simulink model "Cascaded_Rectifier_Isolated_Output"  (R2021b)
settings: Solver=VariableStepAuto  StartTime=0.0  StopTime=0.5  RelTol=1e-3
libraries: spsSeriesRLCBranchLib x41, spsUniversalBridgeLib x28, spsVoltageMeasurementLib x18, spsLinearTransformerLib x8, simulink x8, spsThreeLevelBridgeLib x7, spsACVoltageSourceLib x1, spsCurrentMeasurementLib x1, spsMeanLib x1, slpidlib x1, powerlib_extras x1, spsTHDLib x1
(part 1 of 2)
settings Model: SimulationMode=accelerator  Creator=abc6820292  LastModifiedBy=abc68
settings SolverCC: ZeroCrossAlgorithm=Adaptive
settings DataIOCC: ReturnWorkspaceOutputs=off  Refine=10
settings DebuggingCC: MaskedZcDiagnostic=none  IgnoredZcDiagnostic=none

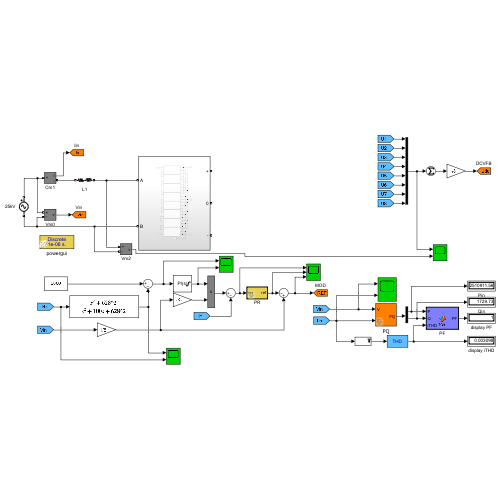
[thumbnail: Simulink's stored preview of the top-level diagram]
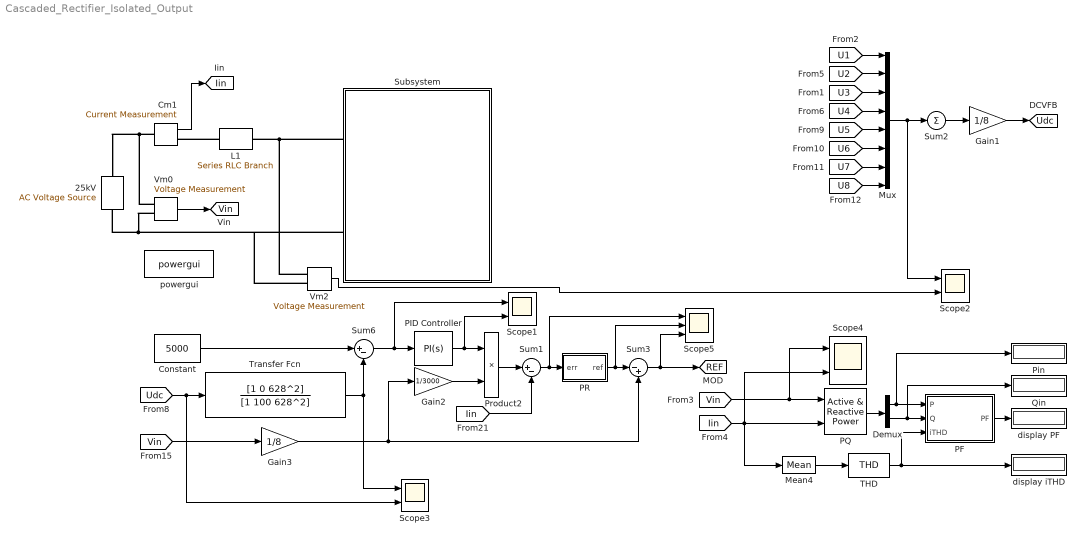
== system Cascaded_Rectifier_Isolated_Output ==
  25kV : spsACVoltageSourceLib/AC Voltage Source  Amplitude=37000  Phase=0  Frequency=50  SampleTime=0  Measurements=None  BusType=swing  Pref=10e3  Qref=0  Qmin=-inf  Qmax=+inf
  Cm1 : spsCurrentMeasurementLib/Current Measurement  PhasorSimulation=off  OutputType=Complex  PSBequivalent=0
  Constant : Constant  Value=5000
  Demux : Demux  Outputs=2
  Gain1 : Gain  Gain=1/8
  Gain2 : Gain  Gain=1/3000
  Gain3 : Gain  Gain=1/8
  L1 : spsSeriesRLCBranchLib/Series RLC Branch  LConnTagsString=__new0  RConnTagsString=__new0  BranchType=RL  Resistance=0.01  Inductance=0.01  SetiL0=off  InitialCurrent=0  Capacitance=inf  Setx0=off  InitialVoltage=0  Measurements=None
  Mean4 : spsMeanLib/Mean  Freq=5000  Vinit=0  Ts=0
  Mux : Mux  Inputs=8
  PF : MATLAB Function  TreatAsAtomicUnit=on
  PID Controller : slpidlib/PID Controller  Controller=PI  Form=Parallel  TimeDomain=Continuous-time  UseExternalTs=off  SampleTime=-1  IntegratorMethod=Forward Euler  FilterMethod=Forward Euler  ControllerParametersSource=internal  P=0.08  I=8  D=0.005  UseFilter=on  N=100  TunerSelectOption=Transfer Function Based (PID Tuner App)  InitialConditionSource=internal  InitialConditionForIntegrator=0  InitialConditionForFilter=0  DifferentiatorICPrevScaledInput=0  ExternalReset=none  TrackingMode=off  Kt=1  LimitOutput=on  SatLimitsSource=internal  UpperSaturationLimit=400  LowerSaturationLimit=-400  LinearizeAsGain=on  AntiWindupMode=clamping  Kb=1  POutMin=[]  POutMax=[]  IOutMin=[]  IOutMax=[]  DOutMin=[]  DOutMax=[]  NOutMin=[]  NOutMax=[]  SumOutMin=[]  SumOutMax=[]  SaturationOutMin=[]  SaturationOutMax=[]  PParamMin=[]  PParamMax=[]  IParamMin=[]  IParamMax=[]  DParamMin=[]  DParamMax=[]  NParamMin=[]  NParamMax=[]  KbParamMin=[]  KbParamMax=[]  KtParamMin=[]  KtParamMax=[]  KbOutMin=[]  KbOutMax=[]  KtOutMin=[]  KtOutMax=[]  IntegratorOutMin=[]  IntegratorOutMax=[]  FilterOutMin=[]  FilterOutMax=[]  SumI1OutMin=[]  SumI1OutMax=[]  SumI2OutMin=[]  SumI2OutMax=[]  SumI3OutMin=[]  SumI3OutMax=[]  SumI4OutMin=[]  SumI4OutMax=[]  SumDOutMin=[]  SumDOutMax=[]  DifferentiatorOutMin=[]  DifferentiatorOutMax=[]  FilterDiffOutCoefMin=[]  FilterDiffOutCoefMax=[]  ReciprocalOutMin=[]  ReciprocalOutMax=[]  SumDenOutMin=[]  SumDenOutMax=[]  SumNumOutMin=[]  SumNumOutMax=[]  DivideOutMin=[]  DivideOutMax=[]  UdiffTsProdOutMin=[]  UdiffTsProdOutMax=[]  NTsProdOutMin=[]  NTsProdOutMax=[]  UintegralTsProdOutMin=[]  UintegralTsProdOutMax=[]  UngainTsProdOutMin=[]  UngainTsProdOutMax=[]  FilterDenConstantOutDataTypeStr=Inherit: Inherit via back propagation  FilterDenConstantOutMin=[]  FilterDenConstantOutMax=[]  PCopyOutDataTypeStr=Inherit: Inherit via back propagation  PCopyOutMin=[]  PCopyOutMax=[]  NCopyOutDataTypeStr=Inherit: Inherit via back propagation  NCopyOutMin=[]  NCopyOutMax=[]  IntegratorContinuousStateAttributes=''  IntegratorStateMustResolveToSignalObject=off  IntegratorRTWStateStorageClass=Auto  FilterContinuousStateAttributes=''  FilterStateMustResolveToSignalObject=off  FilterRTWStateStorageClass=Auto  ParallelPVariant=InternalParameters  IdealPVariant=Disabled  IVariant=InternalParameters  DVariant=Disabled  IntegratorVariant=Continuous  SatVariant=Enabled  AWVariant=ContClampingParallel  PCopyVariant=Disabled  TRVariant=Disabled  FdbkBlocksVariant=Forward  IdealPFdbkVariant=Disabled  SatFdbkVariant=Disabled  DerivativeFilterVariant=Disabled  NVariant=Disabled  NCopyVariant=Disabled_SignalSpec  FilterICVariant=Disabled  IntegratorICVariant=InternalICs  ExternalResetVariant=Disabled  TRSumVariant=Passthrough  SumFdbkVariant=Disabled  SumVariant=Sum_PI  TsampFilterVariant=InternalTs  TsampNgainVariant=Passthrough  TsampIntegralVariant=Passthrough  ExternalSaturationOutDataTypeStr=Inherit: Same as second input
  PQ : powerlib_extras/Measurements/Active & Reactive Power  f1=50
      settings: SourceProductBaseCode=PS
  PR : Subsystem  TreatAsAtomicUnit=on  mask{Kp=12, Kr=1000, Wc=5, Upper=5000, Lower=-5000}
  Pin : Display
      settings: Format=bank
  Product2 : Product  RndMeth=Zero
  Qin : Display
      settings: Format=bank
  Scope{1..4} (4 alike) : Scope  NumInputPorts=2
  Scope5 : Scope  NumInputPorts=3
  Subsystem : Subsystem
  Sum1 : Sum  Inputs=|+-
  Sum2 : Sum  Inputs=+
  Sum3 : Sum  Inputs=|-+
  Sum6 : Sum  Inputs=|+-
  THD : spsTHDLib/THD  Freq=50  Ts=0
      settings: SourceProductBaseCode=PS
  Transfer Fcn : TransferFcn  Numerator=[1 0 628^2]  Denominator=[1 100 628^2]
  Vm0 : spsVoltageMeasurementLib/Voltage Measurement  PhasorSimulation=off  OutputType=Complex  PSBequivalent=0
  Vm2 : spsVoltageMeasurementLib/Voltage Measurement  PhasorSimulation=off  OutputType=Complex  PSBequivalent=0
  display PF : Display
  display iTHD : Display
  powergui : spspowerguiLib/powergui  SimulationMode=Discrete  SampleTime=1e-6  frequency=60  Iterations=50  frequencyindice=0  Pbase=100e6  ErrMax=1e-4  UnitsV=kV  UnitsW=MW  buscounter=0  FunctionMessages=off  echomessages=off  EnableUseOfTLC=off  CurrentSourceSwitches=off  DisableSnubberDevices=off  DisableRonSwitches=off  DisableVfSwitches=off  DisplayEquations=off  AutomaticDiscreteSolvers=off  SolverType=Tustin/Backward Euler (TBE)  Interpol=off  ExternalGateDelay=off  methode=off  Ts=0  x0status=blocks  SPID=off  SwTol=0  HookPort=off  NonlinearTolerance=1e-4  nMaxIteration=100  ContinueOnMaxIteration=off  RestoreLinks=warning  ResistiveCurrentMeasurement=off  Frange=[0:2:500]  Ylog=off  Xlog=on  ShowGrid=off  save=off  variable=ZData  structure=QQQQQ  ZoomFFT=off  StartTime=0.5  cycles=15  DisplayStyle=1  fundamental=50  FreqAxis=off  MaxFrequency=1000  frequencyindicesteady=1  RmsSteady=1  display=off
  tag scope: Iin=global, REF=global, Udc=global, Vin=global
  wires:
  Transfer Fcn/1 -> Sum6/2, Scope3/1
  PF/1(PF) -> display PF/1
  [Iin] -> PQ/2, Scope4/2, Mean4/1
  [Iin] -> Sum1/2
  Sum1/1 -> Scope5/1, PR/1(err)
  Constant/1 -> Sum6/1
  [Vin] -> Scope4/1, PQ/1
  PID Controller/1 -> Product2/1, Scope1/2
  Sum6/1 -> PID Controller/1, Scope1/1
  PR/1(ref) -> Sum3/1, Scope5/2
  PQ/1 -> Demux/1
  Demux/2 -> Qin/1, PF/2(Q)
  THD/1 -> display iTHD/1, PF/3(iTHD)
  Demux/1 -> Pin/1, PF/1(P)
  Product2/1 -> Sum1/1
  Vm0/1 -> [Vin]
  Gain2/1 -> Product2/2
  Cm1/1 -> [Iin]
  Vm2/1 -> Scope2/2
  [U1] -> Mux/1
  [U2] -> Mux/2
  [U3] -> Mux/3
  [U4] -> Mux/4
  Mean4/1 -> THD/1
  [U5] -> Mux/5
  [U6] -> Mux/6
  [U7] -> Mux/7
  [U8] -> Mux/8
  [Udc] -> Scope3/2, Transfer Fcn/1
  Mux/1 -> Scope2/1, Sum2/1
  Sum3/1 -> [REF], Scope5/3
  [Vin] -> Gain3/1
  Gain3/1 -> Sum3/2, Gain2/1
  Sum2/1 -> Gain1/1
  Gain1/1 -> [Udc]
  connections:
  Vm0/LConn2 -- Subsystem/LConn2 -- Vm2/LConn2 -- 25kV/LConn1
  Cm1/LConn1 -- 25kV/RConn1 -- Vm0/LConn1
  L1/LConn1 -- Cm1/RConn1
  Vm2/LConn1 -- Subsystem/LConn1 -- L1/RConn1

== system Cascaded_Rectifier_Isolated_Output/PR ==
  err : Inport
  Kp : Gain  Gain=Kp
  Kr : Gain  Gain=Kr
  Saturation : Saturate  UpperLimit=Upper  LowerLimit=Lower
  Sum3 : Sum  Inputs=|++
  Transfer Fcn : TransferFcn  Numerator=[2*Wc 0]  Denominator=[1 2*Wc 314^2]
  ref : Outport
  wires:
  Kp/1 -> Sum3/1
  Sum3/1 -> Saturation/1
  err/1 -> Kr/1, Kp/1
  Kr/1 -> Transfer Fcn/1
  Transfer Fcn/1 -> Sum3/2
  Saturation/1 -> ref/1

== system Cascaded_Rectifier_Isolated_Output/Subsystem ==
  OFFSET : Constant
  Subsystem1 : Subsystem
      settings: PortSchema="{\"entries\":[{\"content\":{\"sides\":[{\"content\":{\"connectorIds\":[\"LConn1\",\"LConn2\"]},\"type\":\"ConnectorPlacement.EquallySpacedRectSide\",\"uuid\":\"96e89629-64da-437b-b173-a38f2837ffbf\"},{\"content\":{\"connectorIds\":[\"RConn1\",\"In1\",\"RConn2\"],\"side\":\"RIGHT\"},\"type\":\"ConnectorPlacement.EquallySpacedRectSide\",\"uuid\":\"938057d6-1497-4822-9ba7-f8a53ab7498a\"},{\"content\":{\"connectorIds\":[],\"side\":\"TOP\"},\"type\":\"ConnectorPlacement.EquallySpacedRectSide\",\"uuid\":\"796cd648-79ae-42a0-bc56-701f1a02be84\"},{\"content\":{\"connectorIds\":[],\"side\":\"BOTTOM\"},\"type\":\"ConnectorPlacement.EquallySpacedRectSide\",\"uuid\":\"8cf9fed6-175e-4671-8ec7-5c9f69322e59\"}]},\"type\":\"ConnectorPlacement.EquallySpacedConnector\",\"uuid\":\"9c5eea74-f882-4fa8-bc56-80458d0d368f\"}],\"packageUris\":[\"http://schema.mathworks.com/mf0/Connector/R2020b\"],\"version\":\"1.0\"}"
  Subsystem2 : Subsystem
      settings: PortSchema="{\"entries\":[{\"content\":{\"sides\":[{\"content\":{\"connectorIds\":[\"LConn1\",\"LConn2\"]},\"type\":\"ConnectorPlacement.EquallySpacedRectSide\",\"uuid\":\"96e89629-64da-437b-b173-a38f2837ffbf\"},{\"content\":{\"connectorIds\":[\"RConn1\",\"In1\",\"RConn2\"],\"side\":\"RIGHT\"},\"type\":\"ConnectorPlacement.EquallySpacedRectSide\",\"uuid\":\"938057d6-1497-4822-9ba7-f8a53ab7498a\"},{\"content\":{\"connectorIds\":[],\"side\":\"TOP\"},\"type\":\"ConnectorPlacement.EquallySpacedRectSide\",\"uuid\":\"796cd648-79ae-42a0-bc56-701f1a02be84\"},{\"content\":{\"connectorIds\":[],\"side\":\"BOTTOM\"},\"type\":\"ConnectorPlacement.EquallySpacedRectSide\",\"uuid\":\"8cf9fed6-175e-4671-8ec7-5c9f69322e59\"}]},\"type\":\"ConnectorPlacement.EquallySpacedConnector\",\"uuid\":\"9c5eea74-f882-4fa8-bc56-80458d0d368f\"}],\"packageUris\":[\"http://schema.mathworks.com/mf0/Connector/R2020b\"],\"version\":\"1.0\"}"
  Subsystem3 : Subsystem
      settings: PortSchema="{\"entries\":[{\"content\":{\"sides\":[{\"content\":{\"connectorIds\":[\"LConn1\",\"LConn2\"]},\"type\":\"ConnectorPlacement.EquallySpacedRectSide\",\"uuid\":\"96e89629-64da-437b-b173-a38f2837ffbf\"},{\"content\":{\"connectorIds\":[\"RConn1\",\"In1\",\"RConn2\"],\"side\":\"RIGHT\"},\"type\":\"ConnectorPlacement.EquallySpacedRectSide\",\"uuid\":\"938057d6-1497-4822-9ba7-f8a53ab7498a\"},{\"content\":{\"connectorIds\":[],\"side\":\"TOP\"},\"type\":\"ConnectorPlacement.EquallySpacedRectSide\",\"uuid\":\"796cd648-79ae-42a0-bc56-701f1a02be84\"},{\"content\":{\"connectorIds\":[],\"side\":\"BOTTOM\"},\"type\":\"ConnectorPlacement.EquallySpacedRectSide\",\"uuid\":\"8cf9fed6-175e-4671-8ec7-5c9f69322e59\"}]},\"type\":\"ConnectorPlacement.EquallySpacedConnector\",\"uuid\":\"9c5eea74-f882-4fa8-bc56-80458d0d368f\"}],\"packageUris\":[\"http://schema.mathworks.com/mf0/Connector/R2020b\"],\"version\":\"1.0\"}"
  Subsystem4 : Subsystem
      settings: PortSchema="{\"entries\":[{\"content\":{\"sides\":[{\"content\":{\"connectorIds\":[\"LConn1\",\"LConn2\"]},\"type\":\"ConnectorPlacement.EquallySpacedRectSide\",\"uuid\":\"96e89629-64da-437b-b173-a38f2837ffbf\"},{\"content\":{\"connectorIds\":[\"RConn1\",\"In1\",\"RConn2\"],\"side\":\"RIGHT\"},\"type\":\"ConnectorPlacement.EquallySpacedRectSide\",\"uuid\":\"938057d6-1497-4822-9ba7-f8a53ab7498a\"},{\"content\":{\"connectorIds\":[],\"side\":\"TOP\"},\"type\":\"ConnectorPlacement.EquallySpacedRectSide\",\"uuid\":\"796cd648-79ae-42a0-bc56-701f1a02be84\"},{\"content\":{\"connectorIds\":[],\"side\":\"BOTTOM\"},\"type\":\"ConnectorPlacement.EquallySpacedRectSide\",\"uuid\":\"8cf9fed6-175e-4671-8ec7-5c9f69322e59\"}]},\"type\":\"ConnectorPlacement.EquallySpacedConnector\",\"uuid\":\"9c5eea74-f882-4fa8-bc56-80458d0d368f\"}],\"packageUris\":[\"http://schema.mathworks.com/mf0/Connector/R2020b\"],\"version\":\"1.0\"}"
  Subsystem5 : Subsystem
      settings: PortSchema="{\"entries\":[{\"content\":{\"sides\":[{\"content\":{\"connectorIds\":[\"LConn1\",\"LConn2\"]},\"type\":\"ConnectorPlacement.EquallySpacedRectSide\",\"uuid\":\"96e89629-64da-437b-b173-a38f2837ffbf\"},{\"content\":{\"connectorIds\":[\"RConn1\",\"In1\",\"RConn2\"],\"side\":\"RIGHT\"},\"type\":\"ConnectorPlacement.EquallySpacedRectSide\",\"uuid\":\"938057d6-1497-4822-9ba7-f8a53ab7498a\"},{\"content\":{\"connectorIds\":[],\"side\":\"TOP\"},\"type\":\"ConnectorPlacement.EquallySpacedRectSide\",\"uuid\":\"796cd648-79ae-42a0-bc56-701f1a02be84\"},{\"content\":{\"connectorIds\":[],\"side\":\"BOTTOM\"},\"type\":\"ConnectorPlacement.EquallySpacedRectSide\",\"uuid\":\"8cf9fed6-175e-4671-8ec7-5c9f69322e59\"}]},\"type\":\"ConnectorPlacement.EquallySpacedConnector\",\"uuid\":\"9c5eea74-f882-4fa8-bc56-80458d0d368f\"}],\"packageUris\":[\"http://schema.mathworks.com/mf0/Connector/R2020b\"],\"version\":\"1.0\"}"
  Subsystem6 : Subsystem
      settings: PortSchema="{\"entries\":[{\"content\":{\"sides\":[{\"content\":{\"connectorIds\":[\"LConn1\",\"LConn2\"]},\"type\":\"ConnectorPlacement.EquallySpacedRectSide\",\"uuid\":\"96e89629-64da-437b-b173-a38f2837ffbf\"},{\"content\":{\"connectorIds\":[\"RConn1\",\"In1\",\"RConn2\"],\"side\":\"RIGHT\"},\"type\":\"ConnectorPlacement.EquallySpacedRectSide\",\"uuid\":\"938057d6-1497-4822-9ba7-f8a53ab7498a\"},{\"content\":{\"connectorIds\":[],\"side\":\"TOP\"},\"type\":\"ConnectorPlacement.EquallySpacedRectSide\",\"uuid\":\"796cd648-79ae-42a0-bc56-701f1a02be84\"},{\"content\":{\"connectorIds\":[],\"side\":\"BOTTOM\"},\"type\":\"ConnectorPlacement.EquallySpacedRectSide\",\"uuid\":\"8cf9fed6-175e-4671-8ec7-5c9f69322e59\"}]},\"type\":\"ConnectorPlacement.EquallySpacedConnector\",\"uuid\":\"9c5eea74-f882-4fa8-bc56-80458d0d368f\"}],\"packageUris\":[\"http://schema.mathworks.com/mf0/Connector/R2020b\"],\"version\":\"1.0\"}"
  Subsystem7 : Subsystem
      settings: PortSchema="{\"entries\":[{\"content\":{\"sides\":[{\"content\":{\"connectorIds\":[\"LConn1\",\"LConn2\"]},\"type\":\"ConnectorPlacement.EquallySpacedRectSide\",\"uuid\":\"96e89629-64da-437b-b173-a38f2837ffbf\"},{\"content\":{\"connectorIds\":[\"RConn1\",\"In1\",\"RConn2\"],\"side\":\"RIGHT\"},\"type\":\"ConnectorPlacement.EquallySpacedRectSide\",\"uuid\":\"938057d6-1497-4822-9ba7-f8a53ab7498a\"},{\"content\":{\"connectorIds\":[],\"side\":\"TOP\"},\"type\":\"ConnectorPlacement.EquallySpacedRectSide\",\"uuid\":\"796cd648-79ae-42a0-bc56-701f1a02be84\"},{\"content\":{\"connectorIds\":[],\"side\":\"BOTTOM\"},\"type\":\"ConnectorPlacement.EquallySpacedRectSide\",\"uuid\":\"8cf9fed6-175e-4671-8ec7-5c9f69322e59\"}]},\"type\":\"ConnectorPlacement.EquallySpacedConnector\",\"uuid\":\"9c5eea74-f882-4fa8-bc56-80458d0d368f\"}],\"packageUris\":[\"http://schema.mathworks.com/mf0/Connector/R2020b\"],\"version\":\"1.0\"}"
  Subsystem8 : Subsystem
      settings: PortSchema="{\"entries\":[{\"content\":{\"sides\":[{\"content\":{\"connectorIds\":[\"LConn1\",\"LConn2\"]},\"type\":\"ConnectorPlacement.EquallySpacedRectSide\",\"uuid\":\"96e89629-64da-437b-b173-a38f2837ffbf\"},{\"content\":{\"connectorIds\":[\"RConn1\",\"In1\",\"RConn2\"],\"side\":\"RIGHT\"},\"type\":\"ConnectorPlacement.EquallySpacedRectSide\",\"uuid\":\"938057d6-1497-4822-9ba7-f8a53ab7498a\"},{\"content\":{\"connectorIds\":[],\"side\":\"TOP\"},\"type\":\"ConnectorPlacement.EquallySpacedRectSide\",\"uuid\":\"796cd648-79ae-42a0-bc56-701f1a02be84\"},{\"content\":{\"connectorIds\":[],\"side\":\"BOTTOM\"},\"type\":\"ConnectorPlacement.EquallySpacedRectSide\",\"uuid\":\"8cf9fed6-175e-4671-8ec7-5c9f69322e59\"}]},\"type\":\"ConnectorPlacement.EquallySpacedConnector\",\"uuid\":\"9c5eea74-f882-4fa8-bc56-80458d0d368f\"}],\"packageUris\":[\"http://schema.mathworks.com/mf0/Connector/R2020b\"],\"version\":\"1.0\"}"
  A : PMIOPort  Side=Left
  B : PMIOPort  Port=2  Side=Left
  + : PMIOPort  Port=3  Side=Right
  0 : PMIOPort  Port=4  Side=Right
  - : PMIOPort  Port=5  Side=Right
  wires:
  OFFSET/1 -> Subsystem2/1(Idc), Subsystem1/1(Idc), Subsystem3/1(Idc), Subsystem4/1(Idc), Subsystem5/1(Idc), Subsystem6/1(Idc), Subsystem7/1(Idc), Subsystem8/1(Idc)
  connections:
  Subsystem2/LConn1 -- A/RConn1
  Subsystem2/RConn1 -- Subsystem4/RConn1 -- Subsystem3/RConn1 -- Subsystem1/RConn1 -- +/RConn1
  Subsystem2/RConn2 -- 0/RConn1 -- Subsystem4/RConn2 -- Subsystem8/RConn1 -- Subsystem7/RConn1 -- Subsystem6/RConn1 -- Subsystem5/RConn1 -- Subsystem3/RConn2 -- Subsystem1/RConn2
  Subsystem1/LConn1 -- Subsystem2/LConn2
  B/RConn1 -- Subsystem8/LConn2
  Subsystem7/LConn2 -- Subsystem8/LConn1
  Subsystem7/LConn1 -- Subsystem6/LConn2
  Subsystem6/LConn1 -- Subsystem5/LConn2
  Subsystem5/LConn1 -- Subsystem4/LConn2
  Subsystem4/LConn1 -- Subsystem3/LConn2
  Subsystem3/LConn1 -- Subsystem1/LConn2
  Subsystem5/RConn2 -- Subsystem7/RConn2 -- Subsystem8/RConn2 -- -/RConn1 -- Subsystem6/RConn2

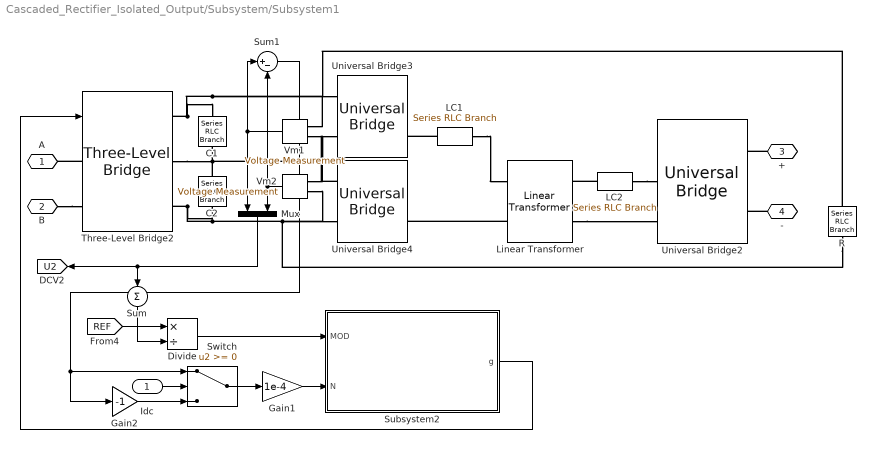
== system Cascaded_Rectifier_Isolated_Output/Subsystem/Subsystem1 ==
  Idc : Inport
  C1 : spsSeriesRLCBranchLib/Series RLC Branch  LConnTagsString=__new0  RConnTagsString=__new0  BranchType=C  Resistance=1  Inductance=7e-4  SetiL0=off  InitialCurrent=0  Capacitance=1e-3  Setx0=on  InitialVoltage=2200  Measurements=None
  C2 : spsSeriesRLCBranchLib/Series RLC Branch  LConnTagsString=__new0  RConnTagsString=__new0  BranchType=C  Resistance=1  Inductance=7e-4  SetiL0=off  InitialCurrent=0  Capacitance=1e-3  Setx0=on  InitialVoltage=2200  Measurements=None
  Divide : Product  Inputs=*/
  Gain1 : Gain  Gain=1e-4
  Gain2 : Gain  Gain=-1
  LC1 : spsSeriesRLCBranchLib/Series RLC Branch  LConnTagsString=__new0  RConnTagsString=__new0  BranchType=LC  Resistance=20  Inductance=2e-5  SetiL0=off  InitialCurrent=0  Capacitance=5.6e-7  Setx0=off  InitialVoltage=0  Measurements=None
  LC2 : spsSeriesRLCBranchLib/Series RLC Branch  LConnTagsString=__new0  RConnTagsString=__new0  BranchType=LC  Resistance=20  Inductance=2e-5  SetiL0=off  InitialCurrent=0  Capacitance=5.6e-7  Setx0=off  InitialVoltage=0  Measurements=None
  Linear Transformer : spsLinearTransformerLib/Linear Transformer  UNITS=SI  NominalPower=[ 250e3 48e3 ]  winding1=[2500 0.01 1e-6]  winding2=[2500 0.01 1e-6]  ThreeWindings=off  winding3=[3.15e+05 0.7938 0.084225]  RmLm=[1e6 1e-4]  Measurements=None  DataType=on
  Mux : Mux  Inputs=2
  R : spsSeriesRLCBranchLib/Series RLC Branch  LConnTagsString=__new0  RConnTagsString=__new0  BranchType=R  Resistance=80  Inductance=7e-4  SetiL0=off  InitialCurrent=0  Capacitance=1e-3  Setx0=off  InitialVoltage=0  Measurements=None
  Subsystem2 : Subsystem
  Sum : Sum  Inputs=+
  Sum1 : Sum  Inputs=|+-
  Switch : Switch
  Three-Level Bridge2 : spsThreeLevelBridgeLib/Three-Level Bridge  Arms=2  SnubberResistance=1e5  SbubberCapacitance=inf  Device=IGBT / Diodes  Ron=1e-3  ForwardVoltages="[  2  2  ]"  Measurements=None
      settings: SourceProductBaseCode=PS
  Universal Bridge2 : spsUniversalBridgeLib/Universal Bridge  Arms=2  SnubberResistance=1e5  SnubberCapacitance=inf  Device=MOSFET / Diodes  Ron=1e-2  Lon=0  ForwardVoltages="[  1  1  ]"  ForwardVoltage=0  GTOparameters=[ 10e-6 , 20e-6 ]  IGBTparameters=[ 1e-6 , 2e-6 ]  Measurements=None  Measurements_2=None  converterType=Rectifier
  Universal Bridge3 : spsUniversalBridgeLib/Universal Bridge  Arms=1  SnubberResistance=1e5  SnubberCapacitance=inf  Device=MOSFET / Diodes  Ron=1e-2  Lon=0  ForwardVoltages="[  1  1  ]"  ForwardVoltage=0  GTOparameters=[ 10e-6 , 20e-6 ]  IGBTparameters=[ 1e-6 , 2e-6 ]  Measurements=None  Measurements_2=None  converterType=Rectifier
  Universal Bridge4 : spsUniversalBridgeLib/Universal Bridge  Arms=1  SnubberResistance=1e5  SnubberCapacitance=inf  Device=MOSFET / Diodes  Ron=1e-2  Lon=0  ForwardVoltages="[  1  1  ]"  ForwardVoltage=0  GTOparameters=[ 10e-6 , 20e-6 ]  IGBTparameters=[ 1e-6 , 2e-6 ]  Measurements=None  Measurements_2=None  converterType=Rectifier
  Vm1 : spsVoltageMeasurementLib/Voltage Measurement  PhasorSimulation=off  OutputType=Complex  PSBequivalent=0
  Vm2 : spsVoltageMeasurementLib/Voltage Measurement  PhasorSimulation=off  OutputType=Complex  PSBequivalent=0
  A : PMIOPort  Side=Left
  B : PMIOPort  Port=2  Side=Left
  + : PMIOPort  Port=3  Side=Right
  - : PMIOPort  Port=4  Side=Right
  tag scope: U2=global
  wires:
  Gain1/1 -> Subsystem2/2(N)
  Sum1/1 -> Switch/1, Gain2/1
  Idc/1 -> Switch/2
  Sum/1 -> Divide/2
  Vm2/1 -> Mux/2, Sum1/2
  Vm1/1 -> Sum1/1, Mux/1
  Mux/1 -> [U2], Sum/1
  Divide/1 -> Subsystem2/1(MOD)
  [REF] -> Divide/1
  Subsystem2/1(g) -> Three-Level Bridge2/1
  Switch/1 -> Gain1/1
  Gain2/1 -> Switch/3
  connections:
  B/RConn1 -- Three-Level Bridge2/LConn2
  Three-Level Bridge2/LConn1 -- A/RConn1
  LC2/LConn1 -- Linear Transformer/RConn1
  LC2/RConn1 -- Universal Bridge2/LConn1
  Linear Transformer/RConn2 -- Universal Bridge2/LConn2
  LC1/RConn1 -- Linear Transformer/LConn1
  Linear Transformer/LConn2 -- Universal Bridge4/LConn1
  LC1/LConn1 -- Universal Bridge3/LConn1
  +/RConn1 -- Universal Bridge2/RConn1
  -/RConn1 -- Universal Bridge2/RConn2
  Three-Level Bridge2/RConn3 -- C2/RConn1 -- Universal Bridge4/RConn2 -- Vm2/LConn2 -- R/RConn1
  Three-Level Bridge2/RConn2 -- C1/RConn1 -- C2/LConn1 -- Universal Bridge4/RConn1 -- Vm2/LConn1 -- Universal Bridge3/RConn2 -- Vm1/LConn2
  Three-Level Bridge2/RConn1 -- Universal Bridge3/RConn1 -- Vm1/LConn1 -- R/LConn1 -- C1/LConn1

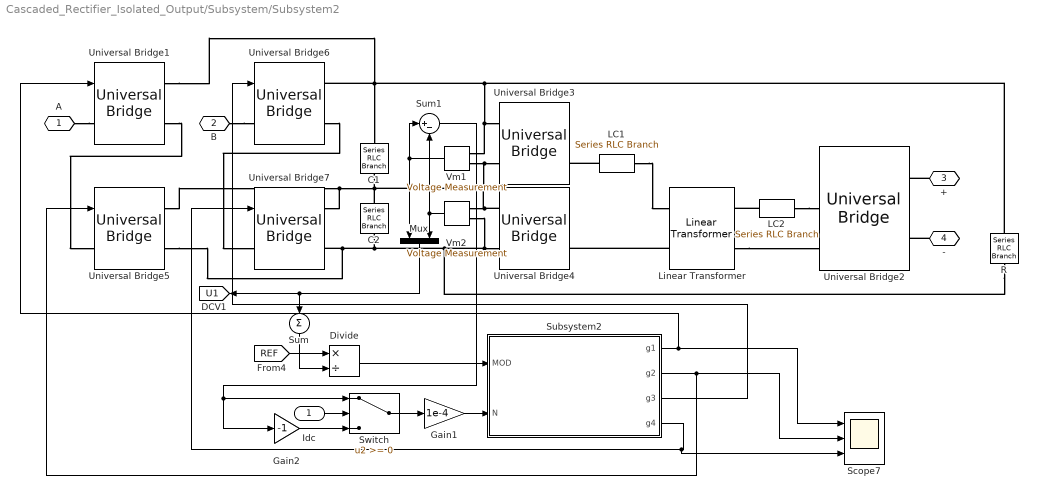
== system Cascaded_Rectifier_Isolated_Output/Subsystem/Subsystem2 ==
  Idc : Inport
  C1 : spsSeriesRLCBranchLib/Series RLC Branch  LConnTagsString=__new0  RConnTagsString=__new0  BranchType=C  Resistance=1  Inductance=7e-4  SetiL0=off  InitialCurrent=0  Capacitance=1e-3  Setx0=on  InitialVoltage=2200  Measurements=None
  C2 : spsSeriesRLCBranchLib/Series RLC Branch  LConnTagsString=__new0  RConnTagsString=__new0  BranchType=C  Resistance=1  Inductance=7e-4  SetiL0=off  InitialCurrent=0  Capacitance=1e-3  Setx0=on  InitialVoltage=2200  Measurements=None
  Divide : Product  Inputs=*/
  Gain1 : Gain  Gain=1e-4
  Gain2 : Gain  Gain=-1
  LC1 : spsSeriesRLCBranchLib/Series RLC Branch  LConnTagsString=__new0  RConnTagsString=__new0  BranchType=LC  Resistance=20  Inductance=2e-5  SetiL0=off  InitialCurrent=0  Capacitance=5.6e-7  Setx0=off  InitialVoltage=0  Measurements=None
  LC2 : spsSeriesRLCBranchLib/Series RLC Branch  LConnTagsString=__new0  RConnTagsString=__new0  BranchType=LC  Resistance=20  Inductance=2e-5  SetiL0=off  InitialCurrent=0  Capacitance=5.6e-7  Setx0=off  InitialVoltage=0  Measurements=None
  Linear Transformer : spsLinearTransformerLib/Linear Transformer  UNITS=SI  NominalPower=[ 250e3 48e3 ]  winding1=[2500 0.01 1e-6]  winding2=[2500 0.01 1e-6]  ThreeWindings=off  winding3=[3.15e+05 0.7938 0.084225]  RmLm=[1e6 1e-4]  Measurements=None  DataType=on
  Mux : Mux  Inputs=2
  R : spsSeriesRLCBranchLib/Series RLC Branch  LConnTagsString=__new0  RConnTagsString=__new0  BranchType=R  Resistance=80  Inductance=7e-4  SetiL0=off  InitialCurrent=0  Capacitance=1e-3  Setx0=off  InitialVoltage=0  Measurements=None
  Scope7 : Scope  NumInputPorts=3
  Subsystem2 : Subsystem
  Sum : Sum  Inputs=+
  Sum1 : Sum  Inputs=|+-
  Switch : Switch
  Universal Bridge{1,5..7} (4 alike) : spsUniversalBridgeLib/Universal Bridge  Arms=1  SnubberResistance=1e5  SnubberCapacitance=inf  Device=IGBT / Diodes  Ron=1e-3  Lon=0  ForwardVoltages="[  2  2  ]"  ForwardVoltage=0  GTOparameters=[ 10e-6 , 20e-6 ]  IGBTparameters=[ 1e-6 , 2e-6 ]  Measurements=None  Measurements_2=None  converterType=Rectifier
  Universal Bridge2 : spsUniversalBridgeLib/Universal Bridge  Arms=2  SnubberResistance=1e5  SnubberCapacitance=inf  Device=MOSFET / Diodes  Ron=1e-2  Lon=0  ForwardVoltages="[  1  1  ]"  ForwardVoltage=0  GTOparameters=[ 10e-6 , 20e-6 ]  IGBTparameters=[ 1e-6 , 2e-6 ]  Measurements=None  Measurements_2=None  converterType=Rectifier
  Universal Bridge3 : spsUniversalBridgeLib/Universal Bridge  Arms=1  SnubberResistance=1e5  SnubberCapacitance=inf  Device=MOSFET / Diodes  Ron=1e-2  Lon=0  ForwardVoltages="[  1  1  ]"  ForwardVoltage=0  GTOparameters=[ 10e-6 , 20e-6 ]  IGBTparameters=[ 1e-6 , 2e-6 ]  Measurements=None  Measurements_2=None  converterType=Rectifier
  Universal Bridge4 : spsUniversalBridgeLib/Universal Bridge  Arms=1  SnubberResistance=1e5  SnubberCapacitance=inf  Device=MOSFET / Diodes  Ron=1e-2  Lon=0  ForwardVoltages="[  1  1  ]"  ForwardVoltage=0  GTOparameters=[ 10e-6 , 20e-6 ]  IGBTparameters=[ 1e-6 , 2e-6 ]  Measurements=None  Measurements_2=None  converterType=Rectifier
  Vm1 : spsVoltageMeasurementLib/Voltage Measurement  PhasorSimulation=off  OutputType=Complex  PSBequivalent=0
  Vm2 : spsVoltageMeasurementLib/Voltage Measurement  PhasorSimulation=off  OutputType=Complex  PSBequivalent=0
  A : PMIOPort  Side=Left
  B : PMIOPort  Port=2  Side=Left
  + : PMIOPort  Port=3  Side=Right
  - : PMIOPort  Port=4  Side=Right
  tag scope: U1=global
  wires:
  Gain2/1 -> Switch/3
  Switch/1 -> Gain1/1
  Subsystem2/1(g1) -> Universal Bridge1/1, Scope7/1
  [REF] -> Divide/1
  Divide/1 -> Subsystem2/1(MOD)
  Mux/1 -> Sum/1, [U1]
  Vm1/1 -> Mux/1, Sum1/1
  Vm2/1 -> Sum1/2, Mux/2
  Sum/1 -> Divide/2
  Idc/1 -> Switch/2
  Sum1/1 -> Switch/1, Gain2/1
  Gain1/1 -> Subsystem2/2(N)
  Subsystem2/2(g2) -> Universal Bridge5/1, Scope7/2
  Subsystem2/3(g3) -> Universal Bridge6/1
  Subsystem2/4(g4) -> Scope7/3, Universal Bridge7/1
  connections:
  Vm1/LConn1 -- Universal Bridge3/RConn1 -- R/LConn1 -- C1/LConn1 -- Universal Bridge1/RConn1 -- Universal Bridge6/RConn1
  C2/LConn1 -- Universal Bridge5/RConn1 -- Universal Bridge7/RConn1 -- Vm1/LConn2 -- Universal Bridge3/RConn2 -- Vm2/LConn1 -- Universal Bridge4/RConn1 -- C1/RConn1
  R/RConn1 -- Vm2/LConn2 -- Universal Bridge4/RConn2 -- Universal Bridge5/RConn2 -- Universal Bridge7/RConn2 -- C2/RConn1
  -/RConn1 -- Universal Bridge2/RConn2
  +/RConn1 -- Universal Bridge2/RConn1
  LC1/LConn1 -- Universal Bridge3/LConn1
  Linear Transformer/LConn2 -- Universal Bridge4/LConn1
  LC1/RConn1 -- Linear Transformer/LConn1
  Linear Transformer/RConn2 -- Universal Bridge2/LConn2
  LC2/RConn1 -- Universal Bridge2/LConn1
  LC2/LConn1 -- Linear Transformer/RConn1
  Universal Bridge1/RConn2 -- Universal Bridge5/LConn1
  A/RConn1 -- Universal Bridge1/LConn1
  Universal Bridge6/RConn2 -- Universal Bridge7/LConn1
  B/RConn1 -- Universal Bridge6/LConn1

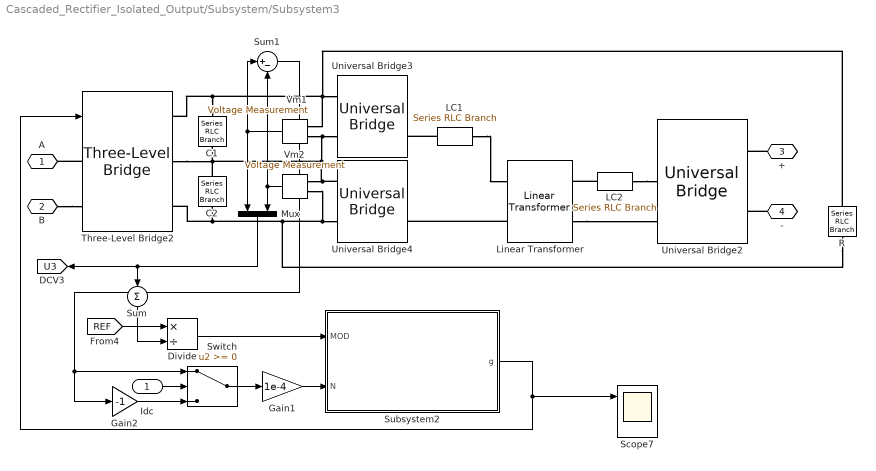
== system Cascaded_Rectifier_Isolated_Output/Subsystem/Subsystem3 ==
  Idc : Inport
  C1 : spsSeriesRLCBranchLib/Series RLC Branch  LConnTagsString=__new0  RConnTagsString=__new0  BranchType=C  Resistance=1  Inductance=7e-4  SetiL0=off  InitialCurrent=0  Capacitance=1e-3  Setx0=on  InitialVoltage=2200  Measurements=None
  C2 : spsSeriesRLCBranchLib/Series RLC Branch  LConnTagsString=__new0  RConnTagsString=__new0  BranchType=C  Resistance=1  Inductance=7e-4  SetiL0=off  InitialCurrent=0  Capacitance=1e-3  Setx0=on  InitialVoltage=2200  Measurements=None
  Divide : Product  Inputs=*/
  Gain1 : Gain  Gain=1e-4
  Gain2 : Gain  Gain=-1
  LC1 : spsSeriesRLCBranchLib/Series RLC Branch  LConnTagsString=__new0  RConnTagsString=__new0  BranchType=LC  Resistance=20  Inductance=2e-5  SetiL0=off  InitialCurrent=0  Capacitance=5.6e-7  Setx0=off  InitialVoltage=0  Measurements=None
  LC2 : spsSeriesRLCBranchLib/Series RLC Branch  LConnTagsString=__new0  RConnTagsString=__new0  BranchType=LC  Resistance=20  Inductance=2e-5  SetiL0=off  InitialCurrent=0  Capacitance=5.6e-7  Setx0=off  InitialVoltage=0  Measurements=None
  Linear Transformer : spsLinearTransformerLib/Linear Transformer  UNITS=SI  NominalPower=[ 250e3 48e3 ]  winding1=[2500 0.01 1e-6]  winding2=[2500 0.01 1e-6]  ThreeWindings=off  winding3=[3.15e+05 0.7938 0.084225]  RmLm=[1e6 1e-4]  Measurements=None  DataType=on
  Mux : Mux  Inputs=2
  R : spsSeriesRLCBranchLib/Series RLC Branch  LConnTagsString=__new0  RConnTagsString=__new0  BranchType=R  Resistance=80  Inductance=7e-4  SetiL0=off  InitialCurrent=0  Capacitance=1e-3  Setx0=off  InitialVoltage=0  Measurements=None
  Scope7 : Scope  NumInputPorts=3
  Subsystem2 : Subsystem
  Sum : Sum  Inputs=+
  Sum1 : Sum  Inputs=|+-
  Switch : Switch
  Three-Level Bridge2 : spsThreeLevelBridgeLib/Three-Level Bridge  Arms=2  SnubberResistance=1e5  SbubberCapacitance=inf  Device=IGBT / Diodes  Ron=1e-3  ForwardVoltages="[  2  2  ]"  Measurements=None
      settings: SourceProductBaseCode=PS
  Universal Bridge2 : spsUniversalBridgeLib/Universal Bridge  Arms=2  SnubberResistance=1e5  SnubberCapacitance=inf  Device=MOSFET / Diodes  Ron=1e-2  Lon=0  ForwardVoltages="[  1  1  ]"  ForwardVoltage=0  GTOparameters=[ 10e-6 , 20e-6 ]  IGBTparameters=[ 1e-6 , 2e-6 ]  Measurements=None  Measurements_2=None  converterType=Rectifier
  Universal Bridge3 : spsUniversalBridgeLib/Universal Bridge  Arms=1  SnubberResistance=1e5  SnubberCapacitance=inf  Device=MOSFET / Diodes  Ron=1e-2  Lon=0  ForwardVoltages="[  1  1  ]"  ForwardVoltage=0  GTOparameters=[ 10e-6 , 20e-6 ]  IGBTparameters=[ 1e-6 , 2e-6 ]  Measurements=None  Measurements_2=None  converterType=Rectifier
  Universal Bridge4 : spsUniversalBridgeLib/Universal Bridge  Arms=1  SnubberResistance=1e5  SnubberCapacitance=inf  Device=MOSFET / Diodes  Ron=1e-2  Lon=0  ForwardVoltages="[  1  1  ]"  ForwardVoltage=0  GTOparameters=[ 10e-6 , 20e-6 ]  IGBTparameters=[ 1e-6 , 2e-6 ]  Measurements=None  Measurements_2=None  converterType=Rectifier
  Vm1 : spsVoltageMeasurementLib/Voltage Measurement  PhasorSimulation=off  OutputType=Complex  PSBequivalent=0
  Vm2 : spsVoltageMeasurementLib/Voltage Measurement  PhasorSimulation=off  OutputType=Complex  PSBequivalent=0
  A : PMIOPort  Side=Left
  B : PMIOPort  Port=2  Side=Left
  + : PMIOPort  Port=3  Side=Right
  - : PMIOPort  Port=4  Side=Right
  tag scope: U3=global
  wires:
  Gain2/1 -> Switch/3
  Switch/1 -> Gain1/1
  Subsystem2/1(g) -> Scope7/1, Three-Level Bridge2/1
  [REF] -> Divide/1
  Divide/1 -> Subsystem2/1(MOD)
  Mux/1 -> Sum/1, [U3]
  Vm1/1 -> Mux/1, Sum1/1
  Vm2/1 -> Sum1/2, Mux/2
  Sum/1 -> Divide/2
  Idc/1 -> Switch/2
  Sum1/1 -> Switch/1, Gain2/1
  Gain1/1 -> Subsystem2/2(N)
  connections:
  C1/LConn1 -- R/LConn1 -- Vm1/LConn1 -- Universal Bridge3/RConn1 -- Three-Level Bridge2/RConn1
  Vm1/LConn2 -- Universal Bridge3/RConn2 -- Vm2/LConn1 -- Universal Bridge4/RConn1 -- C2/LConn1 -- C1/RConn1 -- Three-Level Bridge2/RConn2
  R/RConn1 -- Vm2/LConn2 -- Universal Bridge4/RConn2 -- C2/RConn1 -- Three-Level Bridge2/RConn3
  -/RConn1 -- Universal Bridge2/RConn2
  +/RConn1 -- Universal Bridge2/RConn1
  LC1/LConn1 -- Universal Bridge3/LConn1
  Linear Transformer/LConn2 -- Universal Bridge4/LConn1
  LC1/RConn1 -- Linear Transformer/LConn1
  Linear Transformer/RConn2 -- Universal Bridge2/LConn2
  LC2/RConn1 -- Universal Bridge2/LConn1
  LC2/LConn1 -- Linear Transformer/RConn1
  Three-Level Bridge2/LConn1 -- A/RConn1
  B/RConn1 -- Three-Level Bridge2/LConn2

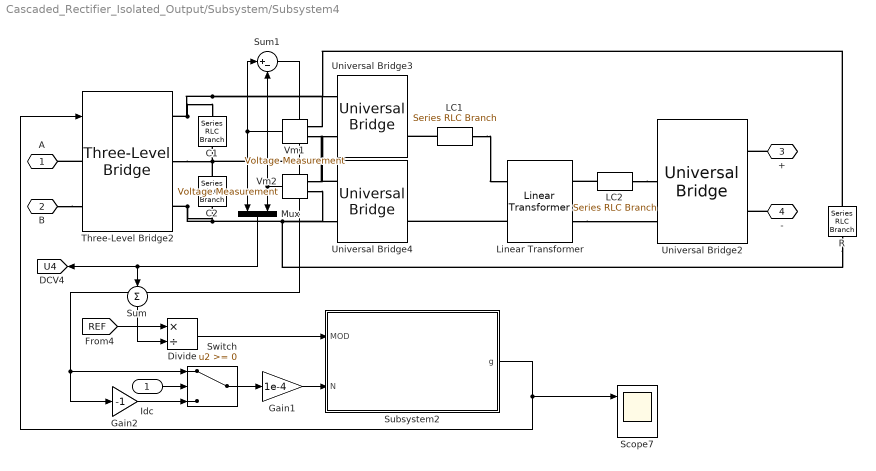
== system Cascaded_Rectifier_Isolated_Output/Subsystem/Subsystem4 ==
  Idc : Inport
  C1 : spsSeriesRLCBranchLib/Series RLC Branch  LConnTagsString=__new0  RConnTagsString=__new0  BranchType=C  Resistance=1  Inductance=7e-4  SetiL0=off  InitialCurrent=0  Capacitance=1e-3  Setx0=on  InitialVoltage=2200  Measurements=None
  C2 : spsSeriesRLCBranchLib/Series RLC Branch  LConnTagsString=__new0  RConnTagsString=__new0  BranchType=C  Resistance=1  Inductance=7e-4  SetiL0=off  InitialCurrent=0  Capacitance=1e-3  Setx0=on  InitialVoltage=2200  Measurements=None
  Divide : Product  Inputs=*/
  Gain1 : Gain  Gain=1e-4
  Gain2 : Gain  Gain=-1
  LC1 : spsSeriesRLCBranchLib/Series RLC Branch  LConnTagsString=__new0  RConnTagsString=__new0  BranchType=LC  Resistance=20  Inductance=2e-5  SetiL0=off  InitialCurrent=0  Capacitance=5.6e-7  Setx0=off  InitialVoltage=0  Measurements=None
  LC2 : spsSeriesRLCBranchLib/Series RLC Branch  LConnTagsString=__new0  RConnTagsString=__new0  BranchType=LC  Resistance=20  Inductance=2e-5  SetiL0=off  InitialCurrent=0  Capacitance=5.6e-7  Setx0=off  InitialVoltage=0  Measurements=None
  Linear Transformer : spsLinearTransformerLib/Linear Transformer  UNITS=SI  NominalPower=[ 250e3 48e3 ]  winding1=[2500 0.01 1e-6]  winding2=[2500 0.01 1e-6]  ThreeWindings=off  winding3=[3.15e+05 0.7938 0.084225]  RmLm=[1e6 1e-4]  Measurements=None  DataType=on
  Mux : Mux  Inputs=2
  R : spsSeriesRLCBranchLib/Series RLC Branch  LConnTagsString=__new0  RConnTagsString=__new0  BranchType=R  Resistance=80  Inductance=7e-4  SetiL0=off  InitialCurrent=0  Capacitance=1e-3  Setx0=off  InitialVoltage=0  Measurements=None
  Scope7 : Scope  NumInputPorts=3
  Subsystem2 : Subsystem
  Sum : Sum  Inputs=+
  Sum1 : Sum  Inputs=|+-
  Switch : Switch
  Three-Level Bridge2 : spsThreeLevelBridgeLib/Three-Level Bridge  Arms=2  SnubberResistance=1e5  SbubberCapacitance=inf  Device=IGBT / Diodes  Ron=1e-3  ForwardVoltages="[  2  2  ]"  Measurements=None
      settings: SourceProductBaseCode=PS
  Universal Bridge2 : spsUniversalBridgeLib/Universal Bridge  Arms=2  SnubberResistance=1e5  SnubberCapacitance=inf  Device=MOSFET / Diodes  Ron=1e-2  Lon=0  ForwardVoltages="[  1  1  ]"  ForwardVoltage=0  GTOparameters=[ 10e-6 , 20e-6 ]  IGBTparameters=[ 1e-6 , 2e-6 ]  Measurements=None  Measurements_2=None  converterType=Rectifier
  Universal Bridge3 : spsUniversalBridgeLib/Universal Bridge  Arms=1  SnubberResistance=1e5  SnubberCapacitance=inf  Device=MOSFET / Diodes  Ron=1e-2  Lon=0  ForwardVoltages="[  1  1  ]"  ForwardVoltage=0  GTOparameters=[ 10e-6 , 20e-6 ]  IGBTparameters=[ 1e-6 , 2e-6 ]  Measurements=None  Measurements_2=None  converterType=Rectifier
  Universal Bridge4 : spsUniversalBridgeLib/Universal Bridge  Arms=1  SnubberResistance=1e5  SnubberCapacitance=inf  Device=MOSFET / Diodes  Ron=1e-2  Lon=0  ForwardVoltages="[  1  1  ]"  ForwardVoltage=0  GTOparameters=[ 10e-6 , 20e-6 ]  IGBTparameters=[ 1e-6 , 2e-6 ]  Measurements=None  Measurements_2=None  converterType=Rectifier
  Vm1 : spsVoltageMeasurementLib/Voltage Measurement  PhasorSimulation=off  OutputType=Complex  PSBequivalent=0
  Vm2 : spsVoltageMeasurementLib/Voltage Measurement  PhasorSimulation=off  OutputType=Complex  PSBequivalent=0
  A : PMIOPort  Side=Left
  B : PMIOPort  Port=2  Side=Left
  + : PMIOPort  Port=3  Side=Right
  - : PMIOPort  Port=4  Side=Right
  tag scope: U4=global
  wires:
  Gain1/1 -> Subsystem2/2(N)
  Sum1/1 -> Switch/1, Gain2/1
  Idc/1 -> Switch/2
  Sum/1 -> Divide/2
  Vm2/1 -> Mux/2, Sum1/2
  Vm1/1 -> Sum1/1, Mux/1
  Mux/1 -> [U4], Sum/1
  Divide/1 -> Subsystem2/1(MOD)
  Subsystem2/1(g) -> Three-Level Bridge2/1, Scope7/1
  Switch/1 -> Gain1/1
  Gain2/1 -> Switch/3
  [REF] -> Divide/1
  connections:
  B/RConn1 -- Three-Level Bridge2/LConn2
  Three-Level Bridge2/LConn1 -- A/RConn1
  LC2/LConn1 -- Linear Transformer/RConn1
  LC2/RConn1 -- Universal Bridge2/LConn1
  Linear Transformer/RConn2 -- Universal Bridge2/LConn2
  LC1/RConn1 -- Linear Transformer/LConn1
  Linear Transformer/LConn2 -- Universal Bridge4/LConn1
  LC1/LConn1 -- Universal Bridge3/LConn1
  +/RConn1 -- Universal Bridge2/RConn1
  -/RConn1 -- Universal Bridge2/RConn2
  Three-Level Bridge2/RConn3 -- C2/RConn1 -- Universal Bridge4/RConn2 -- Vm2/LConn2 -- R/RConn1
  Three-Level Bridge2/RConn2 -- C1/RConn1 -- C2/LConn1 -- Universal Bridge4/RConn1 -- Vm2/LConn1 -- Universal Bridge3/RConn2 -- Vm1/LConn2
  Three-Level Bridge2/RConn1 -- Universal Bridge3/RConn1 -- Vm1/LConn1 -- R/LConn1 -- C1/LConn1

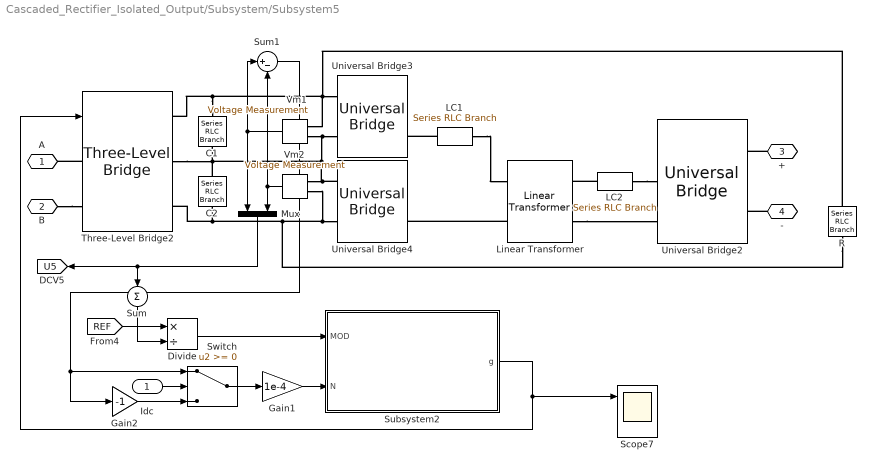
== system Cascaded_Rectifier_Isolated_Output/Subsystem/Subsystem5 ==
  Idc : Inport
  C1 : spsSeriesRLCBranchLib/Series RLC Branch  LConnTagsString=__new0  RConnTagsString=__new0  BranchType=C  Resistance=1  Inductance=7e-4  SetiL0=off  InitialCurrent=0  Capacitance=1e-3  Setx0=on  InitialVoltage=2200  Measurements=None
  C2 : spsSeriesRLCBranchLib/Series RLC Branch  LConnTagsString=__new0  RConnTagsString=__new0  BranchType=C  Resistance=1  Inductance=7e-4  SetiL0=off  InitialCurrent=0  Capacitance=1e-3  Setx0=on  InitialVoltage=2200  Measurements=None
  Divide : Product  Inputs=*/
  Gain1 : Gain  Gain=1e-4
  Gain2 : Gain  Gain=-1
  LC1 : spsSeriesRLCBranchLib/Series RLC Branch  LConnTagsString=__new0  RConnTagsString=__new0  BranchType=LC  Resistance=20  Inductance=2e-5  SetiL0=off  InitialCurrent=0  Capacitance=5.6e-7  Setx0=off  InitialVoltage=0  Measurements=None
  LC2 : spsSeriesRLCBranchLib/Series RLC Branch  LConnTagsString=__new0  RConnTagsString=__new0  BranchType=LC  Resistance=20  Inductance=2e-5  SetiL0=off  InitialCurrent=0  Capacitance=5.6e-7  Setx0=off  InitialVoltage=0  Measurements=None
  Linear Transformer : spsLinearTransformerLib/Linear Transformer  UNITS=SI  NominalPower=[ 250e3 48e3 ]  winding1=[2500 0.01 1e-6]  winding2=[2500 0.01 1e-6]  ThreeWindings=off  winding3=[3.15e+05 0.7938 0.084225]  RmLm=[1e6 1e-4]  Measurements=None  DataType=on
  Mux : Mux  Inputs=2
  R : spsSeriesRLCBranchLib/Series RLC Branch  LConnTagsString=__new0  RConnTagsString=__new0  BranchType=R  Resistance=80  Inductance=7e-4  SetiL0=off  InitialCurrent=0  Capacitance=1e-3  Setx0=off  InitialVoltage=0  Measurements=None
  Scope7 : Scope  NumInputPorts=3
  Subsystem2 : Subsystem
  Sum : Sum  Inputs=+
  Sum1 : Sum  Inputs=|+-
  Switch : Switch
  Three-Level Bridge2 : spsThreeLevelBridgeLib/Three-Level Bridge  Arms=2  SnubberResistance=1e5  SbubberCapacitance=inf  Device=IGBT / Diodes  Ron=1e-3  ForwardVoltages="[  2  2  ]"  Measurements=None
      settings: SourceProductBaseCode=PS
  Universal Bridge2 : spsUniversalBridgeLib/Universal Bridge  Arms=2  SnubberResistance=1e5  SnubberCapacitance=inf  Device=MOSFET / Diodes  Ron=1e-2  Lon=0  ForwardVoltages="[  1  1  ]"  ForwardVoltage=0  GTOparameters=[ 10e-6 , 20e-6 ]  IGBTparameters=[ 1e-6 , 2e-6 ]  Measurements=None  Measurements_2=None  converterType=Rectifier
  Universal Bridge3 : spsUniversalBridgeLib/Universal Bridge  Arms=1  SnubberResistance=1e5  SnubberCapacitance=inf  Device=MOSFET / Diodes  Ron=1e-2  Lon=0  ForwardVoltages="[  1  1  ]"  ForwardVoltage=0  GTOparameters=[ 10e-6 , 20e-6 ]  IGBTparameters=[ 1e-6 , 2e-6 ]  Measurements=None  Measurements_2=None  converterType=Rectifier
  Universal Bridge4 : spsUniversalBridgeLib/Universal Bridge  Arms=1  SnubberResistance=1e5  SnubberCapacitance=inf  Device=MOSFET / Diodes  Ron=1e-2  Lon=0  ForwardVoltages="[  1  1  ]"  ForwardVoltage=0  GTOparameters=[ 10e-6 , 20e-6 ]  IGBTparameters=[ 1e-6 , 2e-6 ]  Measurements=None  Measurements_2=None  converterType=Rectifier
  Vm1 : spsVoltageMeasurementLib/Voltage Measurement  PhasorSimulation=off  OutputType=Complex  PSBequivalent=0
  Vm2 : spsVoltageMeasurementLib/Voltage Measurement  PhasorSimulation=off  OutputType=Complex  PSBequivalent=0
  A : PMIOPort  Side=Left
  B : PMIOPort  Port=2  Side=Left
  + : PMIOPort  Port=3  Side=Right
  - : PMIOPort  Port=4  Side=Right
  tag scope: U5=global
  wires:
  Gain2/1 -> Switch/3
  Switch/1 -> Gain1/1
  Subsystem2/1(g) -> Scope7/1, Three-Level Bridge2/1
  [REF] -> Divide/1
  Divide/1 -> Subsystem2/1(MOD)
  Mux/1 -> Sum/1, [U5]
  Vm1/1 -> Mux/1, Sum1/1
  Vm2/1 -> Sum1/2, Mux/2
  Sum/1 -> Divide/2
  Idc/1 -> Switch/2
  Sum1/1 -> Switch/1, Gain2/1
  Gain1/1 -> Subsystem2/2(N)
  connections:
  C1/LConn1 -- R/LConn1 -- Vm1/LConn1 -- Universal Bridge3/RConn1 -- Three-Level Bridge2/RConn1
  Vm1/LConn2 -- Universal Bridge3/RConn2 -- Vm2/LConn1 -- Universal Bridge4/RConn1 -- C2/LConn1 -- C1/RConn1 -- Three-Level Bridge2/RConn2
  R/RConn1 -- Vm2/LConn2 -- Universal Bridge4/RConn2 -- C2/RConn1 -- Three-Level Bridge2/RConn3
  -/RConn1 -- Universal Bridge2/RConn2
  +/RConn1 -- Universal Bridge2/RConn1
  LC1/LConn1 -- Universal Bridge3/LConn1
  Linear Transformer/LConn2 -- Universal Bridge4/LConn1
  LC1/RConn1 -- Linear Transformer/LConn1
  Linear Transformer/RConn2 -- Universal Bridge2/LConn2
  LC2/RConn1 -- Universal Bridge2/LConn1
  LC2/LConn1 -- Linear Transformer/RConn1
  Three-Level Bridge2/LConn1 -- A/RConn1
  B/RConn1 -- Three-Level Bridge2/LConn2

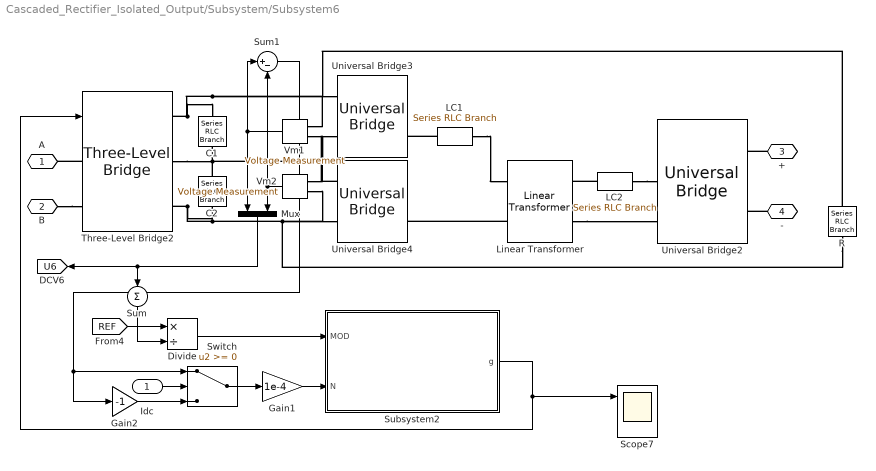
== system Cascaded_Rectifier_Isolated_Output/Subsystem/Subsystem6 ==
  Idc : Inport
  C1 : spsSeriesRLCBranchLib/Series RLC Branch  LConnTagsString=__new0  RConnTagsString=__new0  BranchType=C  Resistance=1  Inductance=7e-4  SetiL0=off  InitialCurrent=0  Capacitance=1e-3  Setx0=on  InitialVoltage=2200  Measurements=None
  C2 : spsSeriesRLCBranchLib/Series RLC Branch  LConnTagsString=__new0  RConnTagsString=__new0  BranchType=C  Resistance=1  Inductance=7e-4  SetiL0=off  InitialCurrent=0  Capacitance=1e-3  Setx0=on  InitialVoltage=2200  Measurements=None
  Divide : Product  Inputs=*/
  Gain1 : Gain  Gain=1e-4
  Gain2 : Gain  Gain=-1
  LC1 : spsSeriesRLCBranchLib/Series RLC Branch  LConnTagsString=__new0  RConnTagsString=__new0  BranchType=LC  Resistance=20  Inductance=2e-5  SetiL0=off  InitialCurrent=0  Capacitance=5.6e-7  Setx0=off  InitialVoltage=0  Measurements=None
  LC2 : spsSeriesRLCBranchLib/Series RLC Branch  LConnTagsString=__new0  RConnTagsString=__new0  BranchType=LC  Resistance=20  Inductance=2e-5  SetiL0=off  InitialCurrent=0  Capacitance=5.6e-7  Setx0=off  InitialVoltage=0  Measurements=None
  Linear Transformer : spsLinearTransformerLib/Linear Transformer  UNITS=SI  NominalPower=[ 250e3 48e3 ]  winding1=[2500 0.01 1e-6]  winding2=[2500 0.01 1e-6]  ThreeWindings=off  winding3=[3.15e+05 0.7938 0.084225]  RmLm=[1e6 1e-4]  Measurements=None  DataType=on
  Mux : Mux  Inputs=2
  R : spsSeriesRLCBranchLib/Series RLC Branch  LConnTagsString=__new0  RConnTagsString=__new0  BranchType=R  Resistance=80  Inductance=7e-4  SetiL0=off  InitialCurrent=0  Capacitance=1e-3  Setx0=off  InitialVoltage=0  Measurements=None
  Scope7 : Scope  NumInputPorts=3
  Subsystem2 : Subsystem
  Sum : Sum  Inputs=+
  Sum1 : Sum  Inputs=|+-
  Switch : Switch
  Three-Level Bridge2 : spsThreeLevelBridgeLib/Three-Level Bridge  Arms=2  SnubberResistance=1e5  SbubberCapacitance=inf  Device=IGBT / Diodes  Ron=1e-3  ForwardVoltages="[  2  2  ]"  Measurements=None
      settings: SourceProductBaseCode=PS
  Universal Bridge2 : spsUniversalBridgeLib/Universal Bridge  Arms=2  SnubberResistance=1e5  SnubberCapacitance=inf  Device=MOSFET / Diodes  Ron=1e-2  Lon=0  ForwardVoltages="[  1  1  ]"  ForwardVoltage=0  GTOparameters=[ 10e-6 , 20e-6 ]  IGBTparameters=[ 1e-6 , 2e-6 ]  Measurements=None  Measurements_2=None  converterType=Rectifier
  Universal Bridge3 : spsUniversalBridgeLib/Universal Bridge  Arms=1  SnubberResistance=1e5  SnubberCapacitance=inf  Device=MOSFET / Diodes  Ron=1e-2  Lon=0  ForwardVoltages="[  1  1  ]"  ForwardVoltage=0  GTOparameters=[ 10e-6 , 20e-6 ]  IGBTparameters=[ 1e-6 , 2e-6 ]  Measurements=None  Measurements_2=None  converterType=Rectifier
  Universal Bridge4 : spsUniversalBridgeLib/Universal Bridge  Arms=1  SnubberResistance=1e5  SnubberCapacitance=inf  Device=MOSFET / Diodes  Ron=1e-2  Lon=0  ForwardVoltages="[  1  1  ]"  ForwardVoltage=0  GTOparameters=[ 10e-6 , 20e-6 ]  IGBTparameters=[ 1e-6 , 2e-6 ]  Measurements=None  Measurements_2=None  converterType=Rectifier
  Vm1 : spsVoltageMeasurementLib/Voltage Measurement  PhasorSimulation=off  OutputType=Complex  PSBequivalent=0
  Vm2 : spsVoltageMeasurementLib/Voltage Measurement  PhasorSimulation=off  OutputType=Complex  PSBequivalent=0
  A : PMIOPort  Side=Left
  B : PMIOPort  Port=2  Side=Left
  + : PMIOPort  Port=3  Side=Right
  - : PMIOPort  Port=4  Side=Right
  tag scope: U6=global
  wires:
  Gain1/1 -> Subsystem2/2(N)
  Sum1/1 -> Switch/1, Gain2/1
  Idc/1 -> Switch/2
  Sum/1 -> Divide/2
  Vm2/1 -> Mux/2, Sum1/2
  Vm1/1 -> Sum1/1, Mux/1
  Mux/1 -> [U6], Sum/1
  Divide/1 -> Subsystem2/1(MOD)
  [REF] -> Divide/1
  Subsystem2/1(g) -> Three-Level Bridge2/1, Scope7/1
  Switch/1 -> Gain1/1
  Gain2/1 -> Switch/3
  connections:
  B/RConn1 -- Three-Level Bridge2/LConn2
  Three-Level Bridge2/LConn1 -- A/RConn1
  LC2/LConn1 -- Linear Transformer/RConn1
  LC2/RConn1 -- Universal Bridge2/LConn1
  Linear Transformer/RConn2 -- Universal Bridge2/LConn2
  LC1/RConn1 -- Linear Transformer/LConn1
  Linear Transformer/LConn2 -- Universal Bridge4/LConn1
  LC1/LConn1 -- Universal Bridge3/LConn1
  +/RConn1 -- Universal Bridge2/RConn1
  -/RConn1 -- Universal Bridge2/RConn2
  Three-Level Bridge2/RConn3 -- C2/RConn1 -- Universal Bridge4/RConn2 -- Vm2/LConn2 -- R/RConn1
  Three-Level Bridge2/RConn2 -- C1/RConn1 -- C2/LConn1 -- Universal Bridge4/RConn1 -- Vm2/LConn1 -- Universal Bridge3/RConn2 -- Vm1/LConn2
  Three-Level Bridge2/RConn1 -- Universal Bridge3/RConn1 -- Vm1/LConn1 -- R/LConn1 -- C1/LConn1

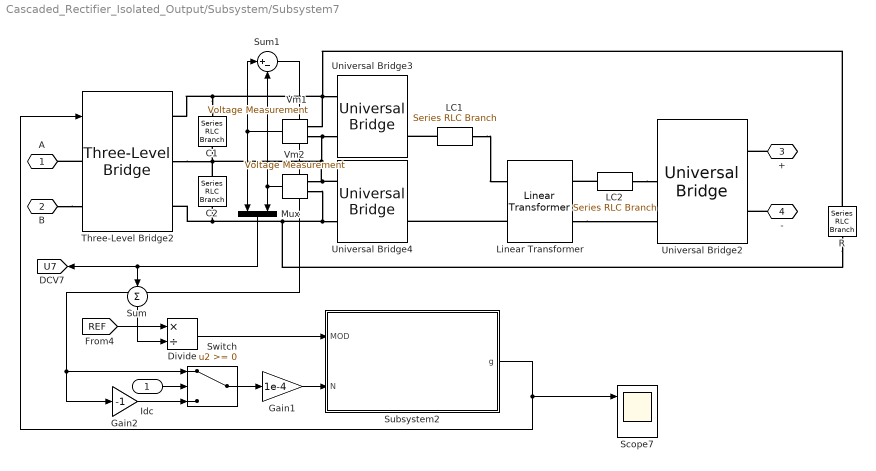
== system Cascaded_Rectifier_Isolated_Output/Subsystem/Subsystem7 ==
  Idc : Inport
  C1 : spsSeriesRLCBranchLib/Series RLC Branch  LConnTagsString=__new0  RConnTagsString=__new0  BranchType=C  Resistance=1  Inductance=7e-4  SetiL0=off  InitialCurrent=0  Capacitance=1e-3  Setx0=on  InitialVoltage=2200  Measurements=None
  C2 : spsSeriesRLCBranchLib/Series RLC Branch  LConnTagsString=__new0  RConnTagsString=__new0  BranchType=C  Resistance=1  Inductance=7e-4  SetiL0=off  InitialCurrent=0  Capacitance=1e-3  Setx0=on  InitialVoltage=2200  Measurements=None
  Divide : Product  Inputs=*/
  Gain1 : Gain  Gain=1e-4
  Gain2 : Gain  Gain=-1
  LC1 : spsSeriesRLCBranchLib/Series RLC Branch  LConnTagsString=__new0  RConnTagsString=__new0  BranchType=LC  Resistance=20  Inductance=2e-5  SetiL0=off  InitialCurrent=0  Capacitance=5.6e-7  Setx0=off  InitialVoltage=0  Measurements=None
  LC2 : spsSeriesRLCBranchLib/Series RLC Branch  LConnTagsString=__new0  RConnTagsString=__new0  BranchType=LC  Resistance=20  Inductance=2e-5  SetiL0=off  InitialCurrent=0  Capacitance=5.6e-7  Setx0=off  InitialVoltage=0  Measurements=None
  Linear Transformer : spsLinearTransformerLib/Linear Transformer  UNITS=SI  NominalPower=[ 250e3 48e3 ]  winding1=[2500 0.01 1e-6]  winding2=[2500 0.01 1e-6]  ThreeWindings=off  winding3=[3.15e+05 0.7938 0.084225]  RmLm=[1e6 1e-4]  Measurements=None  DataType=on
  Mux : Mux  Inputs=2
  R : spsSeriesRLCBranchLib/Series RLC Branch  LConnTagsString=__new0  RConnTagsString=__new0  BranchType=R  Resistance=80  Inductance=7e-4  SetiL0=off  InitialCurrent=0  Capacitance=1e-3  Setx0=off  InitialVoltage=0  Measurements=None
  Scope7 : Scope  NumInputPorts=3
  Subsystem2 : Subsystem
  Sum : Sum  Inputs=+
  Sum1 : Sum  Inputs=|+-
  Switch : Switch
  Three-Level Bridge2 : spsThreeLevelBridgeLib/Three-Level Bridge  Arms=2  SnubberResistance=1e5  SbubberCapacitance=inf  Device=IGBT / Diodes  Ron=1e-3  ForwardVoltages="[  2  2  ]"  Measurements=None
      settings: SourceProductBaseCode=PS
  Universal Bridge2 : spsUniversalBridgeLib/Universal Bridge  Arms=2  SnubberResistance=1e5  SnubberCapacitance=inf  Device=MOSFET / Diodes  Ron=1e-2  Lon=0  ForwardVoltages="[  1  1  ]"  ForwardVoltage=0  GTOparameters=[ 10e-6 , 20e-6 ]  IGBTparameters=[ 1e-6 , 2e-6 ]  Measurements=None  Measurements_2=None  converterType=Rectifier
  Universal Bridge3 : spsUniversalBridgeLib/Universal Bridge  Arms=1  SnubberResistance=1e5  SnubberCapacitance=inf  Device=MOSFET / Diodes  Ron=1e-2  Lon=0  ForwardVoltages="[  1  1  ]"  ForwardVoltage=0  GTOparameters=[ 10e-6 , 20e-6 ]  IGBTparameters=[ 1e-6 , 2e-6 ]  Measurements=None  Measurements_2=None  converterType=Rectifier
  Universal Bridge4 : spsUniversalBridgeLib/Universal Bridge  Arms=1  SnubberResistance=1e5  SnubberCapacitance=inf  Device=MOSFET / Diodes  Ron=1e-2  Lon=0  ForwardVoltages="[  1  1  ]"  ForwardVoltage=0  GTOparameters=[ 10e-6 , 20e-6 ]  IGBTparameters=[ 1e-6 , 2e-6 ]  Measurements=None  Measurements_2=None  converterType=Rectifier
  Vm1 : spsVoltageMeasurementLib/Voltage Measurement  PhasorSimulation=off  OutputType=Complex  PSBequivalent=0
  Vm2 : spsVoltageMeasurementLib/Voltage Measurement  PhasorSimulation=off  OutputType=Complex  PSBequivalent=0
  A : PMIOPort  Side=Left
  B : PMIOPort  Port=2  Side=Left
  + : PMIOPort  Port=3  Side=Right
  - : PMIOPort  Port=4  Side=Right
  tag scope: U7=global
  wires:
  Gain2/1 -> Switch/3
  Switch/1 -> Gain1/1
  Subsystem2/1(g) -> Scope7/1, Three-Level Bridge2/1
  [REF] -> Divide/1
  Divide/1 -> Subsystem2/1(MOD)
  Mux/1 -> Sum/1, [U7]
  Vm1/1 -> Mux/1, Sum1/1
  Vm2/1 -> Sum1/2, Mux/2
  Sum/1 -> Divide/2
  Idc/1 -> Switch/2
  Sum1/1 -> Switch/1, Gain2/1
  Gain1/1 -> Subsystem2/2(N)
  connections:
  C1/LConn1 -- R/LConn1 -- Vm1/LConn1 -- Universal Bridge3/RConn1 -- Three-Level Bridge2/RConn1
  Vm1/LConn2 -- Universal Bridge3/RConn2 -- Vm2/LConn1 -- Universal Bridge4/RConn1 -- C2/LConn1 -- C1/RConn1 -- Three-Level Bridge2/RConn2
  R/RConn1 -- Vm2/LConn2 -- Universal Bridge4/RConn2 -- C2/RConn1 -- Three-Level Bridge2/RConn3
  -/RConn1 -- Universal Bridge2/RConn2
  +/RConn1 -- Universal Bridge2/RConn1
  LC1/LConn1 -- Universal Bridge3/LConn1
  Linear Transformer/LConn2 -- Universal Bridge4/LConn1
  LC1/RConn1 -- Linear Transformer/LConn1
  Linear Transformer/RConn2 -- Universal Bridge2/LConn2
  LC2/RConn1 -- Universal Bridge2/LConn1
  LC2/LConn1 -- Linear Transformer/RConn1
  Three-Level Bridge2/LConn1 -- A/RConn1
  B/RConn1 -- Three-Level Bridge2/LConn2
